simulink library "Damper_Control_dCoeff"  (R2025a)
settings: Solver=VariableStepAuto  StartTime=0.0  StopTime=10.0  RelTol=1e-3
undefined symbols (not defined in the file or in its folder): Control
libraries: Vehicle_Inputs x1, Vehicle_Outputs x1
Description:
  | Copyright 2026 The MathWorks, Inc.
settings Model: Creator=smiller  LastModifiedBy=smiller
settings OptimizationCC: ReuseModelBlockBuffer=off
settings ModelReferenceCC: EnableRefExpFcnMdlSchedulingChecks=on
settings RTWCC: GPUComputeCapability=3.5

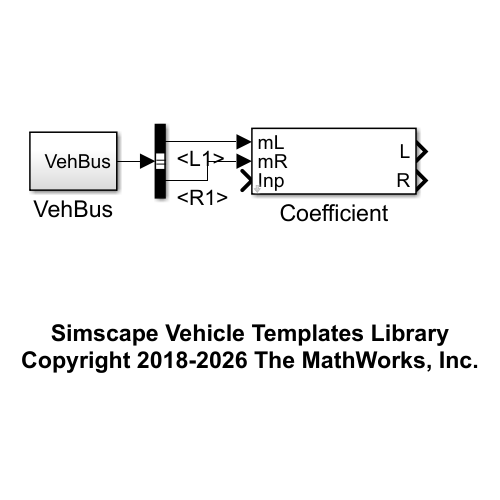
[thumbnail: Simulink's stored preview of the top-level diagram]
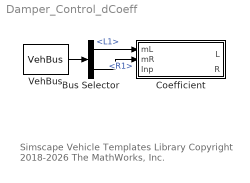
== system Damper_Control_dCoeff ==
  note: Simscape Vehicle Templates Library
      | Copyright 2018-2026 The MathWorks, Inc.
  Bus Selector : BusSelector  OutputSignals=Chassis.Damper.L1,Chassis.Damper.R1
  Coefficient : Subsystem  mask(Control Law for Damper Coefficient){b_A1=Control.Damper.Axle1.tFilt, brkPts_dim1_A1=Control.Damper.Axle1.vDamperd, brkPts_dim2_A1=Control.Damper.Axle1.iControl, Table_A1=Control.Damper.Axle1.dDamper}
      mask prompts: b_A1 "Filter time constant (sec)"; brkPts_dim1_A1 "Damper Speed [1xm] (m/s)"; brkPts_dim2_A1 "Input 2 [1xn] (1)"; Table_A1 "Damper Coefficient [mxn] (N/(m/s))"
      mask help: Determines damping coefficient based on damper speed and a second input signal.
      mask TypeOptions b_A1: Filter/b
      mask TypeOptions brkPts_dim1_A1: Lookup Table Coeff/BreakpointsForDimension1
      mask TypeOptions brkPts_dim2_A1: Lookup Table Coeff/BreakpointsForDimension2
      mask TypeOptions Table_A1: Lookup Table Coeff/Table
      mask DialogControl cont_axle1 Prompt: Axle 1
  VehBus : Vehicle_Outputs/VehBus  SystemSampleTime=-1  VariantActivationTime=update diagram  EmptyChoice=off  PassThrough=off  PassThroughVariantControl=(default)  EmptyChoiceVariantControl=(default)  AllowFlexibleInterface=on  Latency=0  AutoFrameSizeCalculation=off
  wires:
  Bus Selector/2 -> Coefficient/2(mR)  "<R1>"
  VehBus/1 -> Bus Selector/1
  Bus Selector/1 -> Coefficient/1(mL)  "<L1>"

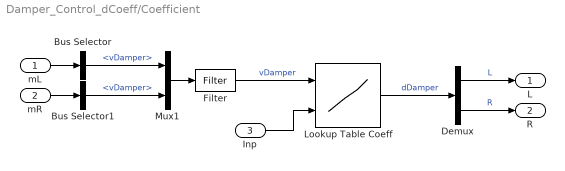
== system Damper_Control_dCoeff/Coefficient ==
  mL : Inport
  mR : Inport  Port=2
  Inp : Inport  Port=3
  Bus Selector : BusSelector  OutputSignals=vDamper
  Bus Selector1 : BusSelector  OutputSignals=vDamper
  Demux : Demux  Outputs=2
  Filter : Vehicle_Inputs/Filter  b=b_A1  x_initial=[0 0]
  Lookup Table Coeff : Lookup_n-D  BreakpointsForDimension1=brkPts_dim1_A1  BreakpointsForDimension2=brkPts_dim2_A1  Table=Table_A1  InternalRulePriority=Speed  RndMeth=Simplest
      settings: InputPortMap=u0,u1
  Mux1 : Mux  Inputs=2
  L : Outport  VectorParamsAs1DForOutWhenUnconnected=off
  R : Outport  Port=2  VectorParamsAs1DForOutWhenUnconnected=off
  wires:
  Lookup Table Coeff/1 -> Demux/1  "dDamper"
  Inp/1 -> Lookup Table Coeff/2
  Demux/2 -> R/1  "R"
  Demux/1 -> L/1  "L"
  Mux1/1 -> Filter/1
  Bus Selector/1 -> Mux1/1  "<vDamper>"
  Filter/1 -> Lookup Table Coeff/1  "vDamper"
  mL/1 -> Bus Selector/1
  mR/1 -> Bus Selector1/1
  Bus Selector1/1 -> Mux1/2  "<vDamper>"
